simulink model "Pushbutton_to_PWMv2"  (Simulink 7.6)
settings: Solver=FixedStepDiscrete  SolverMode=SingleTasking  StartTime=0.0  StopTime=inf  FixedStep=.0001  RelTol=1e-3
undefined symbols (not defined in the file or in its folder): OC2max
libraries: simulink x16, dsPICdrivers x9, dspswit3 x1
settings Model: Creator=ij8977  LastModifiedBy=ij8977  ExtModeTrigDuration=10000
settings SolverCC: PositivePriorityOrder=on
settings OptimizationCC: OptimizeModelRefInitCode=on  LifeSpan=Inf
settings DebuggingCC: StrictBusMsg=Warning
settings RTWCC: SystemTargetFile=pic32.tlc  MakeCommand=make_CreateMPLAB  TemplateMakefile=pic32_gcc.tmf  PostCodeGenCommand=dsPIC_Compile()  Description=Embedded Target for Microchip dsPIC (real-time)  ProcessScript=pic32_make_rtw_hook
settings CodeAppCC: IgnoreCustomStorageClasses=off
settings STFCustomTargetCC: IncludeMdlTerminateFcn=off  CombineOutputUpdateFcns=on  SuppressErrorStatus=on  ERTCustomFileBanners=on  SupportContinuousTime=off  SupportNonInlinedSFcns=off  SystemTargetFile=pic32.tlc
settings ERTTargetCC: MultiwordLength=2048  ParMdlRefBuildCompliant=off  CompOptLevelCompliant=off  IncludeMdlTerminateFcn=off  SuppressErrorStatus=on  ERTFirstTimeCompliant=off  ModelStepFunctionPrototypeControlCompliant=off  CPPClassGenCompliant=off  InlinedParameterPlacement=NonHierarchical  ERTSrcFileBannerTemplate=dsPIC_code_template.cgt  ERTHdrFileBannerTemplate=dsPIC_code_template.cgt  ERTDataSrcFileTemplate=dsPIC_code_template.cgt  ERTDataHdrFileTemplate=dsPIC_code_template.cgt  ERTCustomFileTemplate=dsPIC_main.tlc  ConvertIfToSwitch=off
settings CustomProperty: DataType=string  Value=C:\PROGRA~1\MATLAB\R2010b\bin\win32\gmake

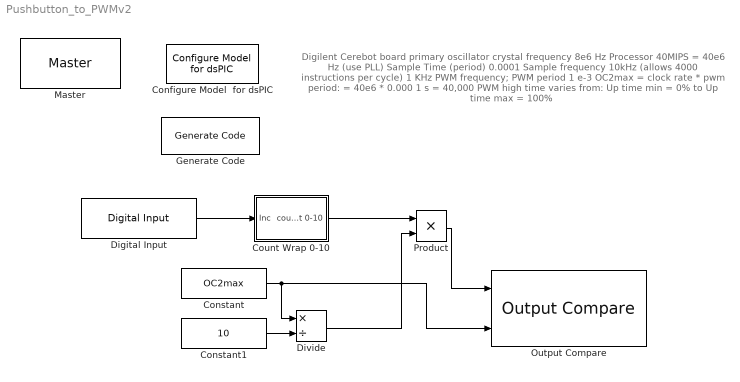
== system Pushbutton_to_PWMv2 ==
  note: Digilent Cerebot board primary oscillator crystal frequency 8e6 Hz
      | Processor 40MIPS = 40e6 Hz (use PLL)
      | Sample Time (period) 0.0001   Sample frequency 10kHz (allows 4000 instructions per cycle)
      | 1 KHz PWM frequency; PWM period 1 e-3
      | OC2max = clock rate * pwm period: = 40e6 * 0.000 1 s = 40,000
      | PWM high time varies from:
      | Up time min = 0%
      | to
      | Up time max = 100%
  Configure Model  for dsPIC : dsPICdrivers/Simulink Configuration/Configure Model  for dsPIC
  Constant : Constant  Value=OC2max  OutDataTypeStr=uint16
  Constant1 : Constant  Value=10  OutDataTypeStr=uint16
  Count Wrap 0-10 : Subsystem
  Digital Input : dsPICdrivers/Digital I//O/Digital Input  Tag=dsPIC_Digital_Input  PORT=A  Pin=[6]  SampleTime=.0001  OrderingInOutPopup=None
  Divide : Product  Inputs=*/
  Generate Code : dsPICdrivers/Simulink Configuration/Generate Code
  Master : dsPICdrivers/Master  Tag=dsPIC_MASTER  Priority=1  TimeStepType=Timer1  picType=32MX460F512L  fcy=40000000  Quartz_33f=8e6  PLLActive_33f=on  fcyDesired_33f=40e6  tmr1="[1  3999  0]"  tmr1Info="Time Step : 0.0001  ;   Error : 0%  PR1=3999"  tmr2345="[1  0  0  0]"  tmr2345cfg=[-1 -1 -1 -1]  IOautoConf=on  typePort="[ 0   0   0   0   0   0   9   0   0   0   0   0   0   0   0   0   0   0   0   0   0   0   0   0   0   0  10  10  10  10   0   0   0   0   0   0   0   0   0   0   0   0   0   0   0   0   0   0   0   7   0   0   0   0   0   0   0   0   0   0   0   0   0   0   0   0   0   0   0   0   0   0   0   0   0   0   0   0   0   0   0   0   0   0   0   0   0   0   0   0   0   0   0   0   0   0   0   0   0   0   0   0   0   0   0   0   0   0   0   0   0   0 ]"  TRIS="[ 65535  50175  65535  65533  65535  65535  65535 ]"  ADPCFG=15360  MasterBusyPort=None  MasterOverloadPort=None  FOSC=Quartz (XT - HS)  ClockSwitchMonitor=Both disabled  TempProtection_33f=TEMP_ON  FPBOR=<empty>  PWRT=disable  MCLR=<empty>  ICD=ICS_PGD1  JTAGEN=JTAGEN_OFF  PowerSave=off  OverrideFcy=off  NewFcy=1e6  PR2345="[65535  65535  65535  65535]"
  Output Compare : dsPICdrivers/Peripheral I//O/Output Compare  Tag=dsPIC_PWM_out  Priority=5  IntPriority=3  CHANNEL=[2]  Channel_UP_Down_Periode=[5]  MaxChannel=[0.001]  MaxName=' OC2max '  Precision=[15.2876]  Timer=[2]  Status=OK  SafeMarge=[0]  PortLetter=[68]  PortNumber=[1]  MaxValues=[39999]
  Product : Product  OutDataTypeStr=uint16  RndMeth=Zero
  wires:
  Digital Input/1 -> Count Wrap 0-10/1(Inc)
  Count Wrap 0-10/1(count 0-10) -> Product/1
  Constant1/1 -> Divide/2
  Constant/1 -> Divide/1, Output Compare/2
  Product/1 -> Output Compare/1
  Divide/1 -> Product/2

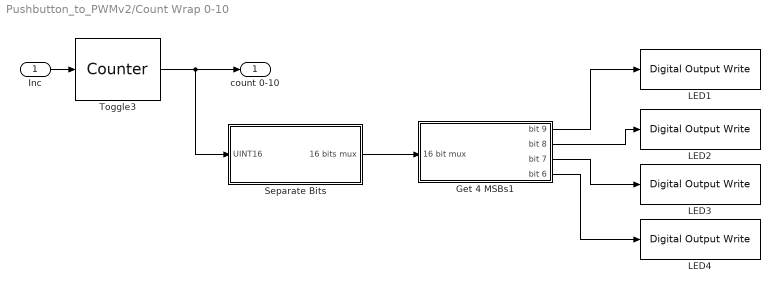
== system Pushbutton_to_PWMv2/Count Wrap 0-10 ==
  Inc : Inport
  Get 4 MSBs1 : Subsystem
  LED1 : dsPICdrivers/Digital I//O/Digital Output Write  Tag=dsPIC_Digital_Output  Priority=5  PORT=B  Pin=[10]  Simultaneous=off  OrderingInOutPopup=None
  LED2 : dsPICdrivers/Digital I//O/Digital Output Write  Tag=dsPIC_Digital_Output  Priority=5  PORT=B  Pin=[11]  Simultaneous=off  OrderingInOutPopup=None
  LED3 : dsPICdrivers/Digital I//O/Digital Output Write  Tag=dsPIC_Digital_Output  Priority=5  PORT=B  Pin=[12]  Simultaneous=off  OrderingInOutPopup=None
  LED4 : dsPICdrivers/Digital I//O/Digital Output Write  Tag=dsPIC_Digital_Output  Priority=5  PORT=B  Pin=[13]  Simultaneous=off  OrderingInOutPopup=None
  Separate Bits : Subsystem
  Toggle3 : dspswit3/Counter  Direction=Up  CountEvent=Rising edge  CounterSize=User defined  MaxCount=10  InitialCount=0  Output=Count  HitValue=10  ResetInput=off  SamplesPerFrame=1  Ts=1  CntDtype=uint16  HitDtype=Logical
  count 0-10 : Outport
  wires:
  Inc/1 -> Toggle3/1
  Get 4 MSBs1/1(bit 9) -> LED1/1
  Get 4 MSBs1/2(bit 8) -> LED2/1
  Get 4 MSBs1/3(bit 7) -> LED3/1
  Get 4 MSBs1/4(bit 6) -> LED4/1
  Separate Bits/1(16 bits mux) -> Get 4 MSBs1/1(16 bit mux)
  Toggle3/1 -> count 0-10/1, Separate Bits/1(UINT16)

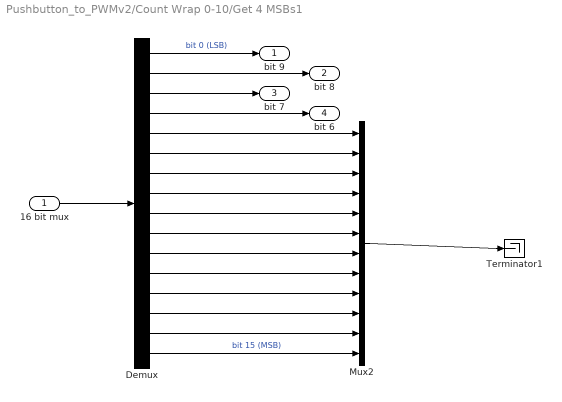
== system Pushbutton_to_PWMv2/Count Wrap 0-10/Get 4 MSBs1 ==
  16 bit mux : Inport  OutDataTypeStr=boolean
  Demux : Demux  Outputs=16
  Mux2 : Mux  Inputs=12
  Terminator1 : Terminator
  bit 9 : Outport
  bit 8 : Outport  Port=2
  bit 7 : Outport  Port=3
  bit 6 : Outport  Port=4
  wires:
  16 bit mux/1 -> Demux/1
  Mux2/1 -> Terminator1/1
  Demux/4 -> bit 6/1
  Demux/3 -> bit 7/1
  Demux/2 -> bit 8/1
  Demux/1 -> bit 9/1  "bit 0 (LSB)"
  Demux/5 -> Mux2/1
  Demux/6 -> Mux2/2
  Demux/7 -> Mux2/3
  Demux/8 -> Mux2/4
  Demux/9 -> Mux2/5
  Demux/10 -> Mux2/6
  Demux/11 -> Mux2/7
  Demux/12 -> Mux2/8
  Demux/13 -> Mux2/9
  Demux/14 -> Mux2/10
  Demux/15 -> Mux2/11
  Demux/16 -> Mux2/12  "bit 15 (MSB)"

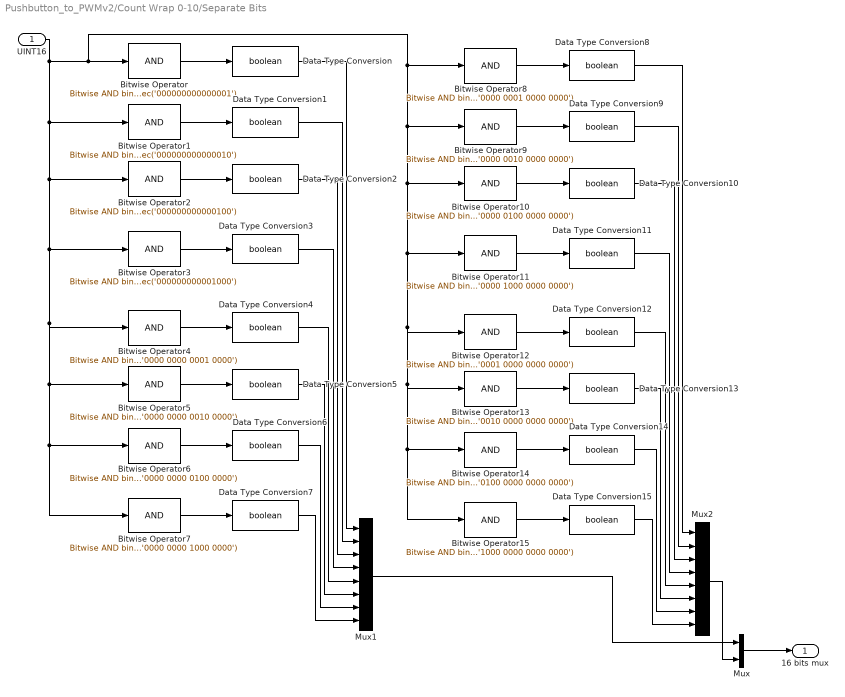
== system Pushbutton_to_PWMv2/Count Wrap 0-10/Separate Bits ==
  UINT16 : Inport
  Bitwise Operator : simulink/Logic and Bit Operations/Bitwise Operator  logicop=AND  UseBitMask=on  BitMask=bin2dec('000000000000001')  BitMaskRealWorld=Stored Integer
  Bitwise Operator1 : simulink/Logic and Bit Operations/Bitwise Operator  logicop=AND  UseBitMask=on  BitMask=bin2dec('000000000000010')  BitMaskRealWorld=Stored Integer
  Bitwise Operator10 : simulink/Logic and Bit Operations/Bitwise Operator  logicop=AND  UseBitMask=on  BitMask=bin2dec('0000 0100 0000 0000')  BitMaskRealWorld=Stored Integer
  Bitwise Operator11 : simulink/Logic and Bit Operations/Bitwise Operator  logicop=AND  UseBitMask=on  BitMask=bin2dec('0000 1000 0000 0000')  BitMaskRealWorld=Stored Integer
  Bitwise Operator12 : simulink/Logic and Bit Operations/Bitwise Operator  logicop=AND  UseBitMask=on  BitMask=bin2dec('0001 0000 0000 0000')  BitMaskRealWorld=Stored Integer
  Bitwise Operator13 : simulink/Logic and Bit Operations/Bitwise Operator  logicop=AND  UseBitMask=on  BitMask=bin2dec('0010 0000 0000 0000')  BitMaskRealWorld=Stored Integer
  Bitwise Operator14 : simulink/Logic and Bit Operations/Bitwise Operator  logicop=AND  UseBitMask=on  BitMask=bin2dec('0100 0000 0000 0000')  BitMaskRealWorld=Stored Integer
  Bitwise Operator15 : simulink/Logic and Bit Operations/Bitwise Operator  logicop=AND  UseBitMask=on  BitMask=bin2dec('1000 0000 0000 0000')  BitMaskRealWorld=Stored Integer
  Bitwise Operator2 : simulink/Logic and Bit Operations/Bitwise Operator  logicop=AND  UseBitMask=on  BitMask=bin2dec('000000000000100')  BitMaskRealWorld=Stored Integer
  Bitwise Operator3 : simulink/Logic and Bit Operations/Bitwise Operator  logicop=AND  UseBitMask=on  BitMask=bin2dec('000000000001000')  BitMaskRealWorld=Stored Integer
  Bitwise Operator4 : simulink/Logic and Bit Operations/Bitwise Operator  logicop=AND  UseBitMask=on  BitMask=bin2dec('0000 0000 0001 0000')  BitMaskRealWorld=Stored Integer
  Bitwise Operator5 : simulink/Logic and Bit Operations/Bitwise Operator  logicop=AND  UseBitMask=on  BitMask=bin2dec('0000 0000 0010 0000')  BitMaskRealWorld=Stored Integer
  Bitwise Operator6 : simulink/Logic and Bit Operations/Bitwise Operator  logicop=AND  UseBitMask=on  BitMask=bin2dec('0000 0000 0100 0000')  BitMaskRealWorld=Stored Integer
  Bitwise Operator7 : simulink/Logic and Bit Operations/Bitwise Operator  logicop=AND  UseBitMask=on  BitMask=bin2dec('0000 0000 1000 0000')  BitMaskRealWorld=Stored Integer
  Bitwise Operator8 : simulink/Logic and Bit Operations/Bitwise Operator  logicop=AND  UseBitMask=on  BitMask=bin2dec('0000 0001 0000 0000')  BitMaskRealWorld=Stored Integer
  Bitwise Operator9 : simulink/Logic and Bit Operations/Bitwise Operator  logicop=AND  UseBitMask=on  BitMask=bin2dec('0000 0010 0000 0000')  BitMaskRealWorld=Stored Integer
  Data Type Conversion{,1..15} (16 alike) : DataTypeConversion  OutDataTypeStr=boolean
  Mux : Mux  Inputs=2
  Mux1 : Mux  Inputs=8
  Mux2 : Mux  Inputs=8
  16 bits mux : Outport
  wires:
  Mux2/1 -> Mux/2
  Bitwise Operator15/1 -> Data Type Conversion15/1
  Bitwise Operator14/1 -> Data Type Conversion14/1
  Bitwise Operator13/1 -> Data Type Conversion13/1
  Bitwise Operator12/1 -> Data Type Conversion12/1
  Bitwise Operator11/1 -> Data Type Conversion11/1
  Bitwise Operator10/1 -> Data Type Conversion10/1
  Bitwise Operator9/1 -> Data Type Conversion9/1
  Data Type Conversion15/1 -> Mux2/8
  Data Type Conversion14/1 -> Mux2/7
  Data Type Conversion13/1 -> Mux2/6
  Data Type Conversion12/1 -> Mux2/5
  Data Type Conversion11/1 -> Mux2/4
  Data Type Conversion10/1 -> Mux2/3
  Data Type Conversion9/1 -> Mux2/2
  Data Type Conversion8/1 -> Mux2/1
  Bitwise Operator8/1 -> Data Type Conversion8/1
  Bitwise Operator7/1 -> Data Type Conversion7/1
  Bitwise Operator6/1 -> Data Type Conversion6/1
  Bitwise Operator5/1 -> Data Type Conversion5/1
  Bitwise Operator4/1 -> Data Type Conversion4/1
  Bitwise Operator3/1 -> Data Type Conversion3/1
  Bitwise Operator2/1 -> Data Type Conversion2/1
  Bitwise Operator1/1 -> Data Type Conversion1/1
  Mux/1 -> 16 bits mux/1
  Mux1/1 -> Mux/1
  Data Type Conversion7/1 -> Mux1/8
  Data Type Conversion6/1 -> Mux1/7
  Data Type Conversion5/1 -> Mux1/6
  Data Type Conversion4/1 -> Mux1/5
  Data Type Conversion3/1 -> Mux1/4
  Data Type Conversion2/1 -> Mux1/3
  Data Type Conversion1/1 -> Mux1/2
  Data Type Conversion/1 -> Mux1/1
  Bitwise Operator/1 -> Data Type Conversion/1
  UINT16/1 -> Bitwise Operator8/1, Bitwise Operator9/1, Bitwise Operator10/1, Bitwise Operator11/1, Bitwise Operator12/1, Bitwise Operator13/1, Bitwise Operator14/1, Bitwise Operator15/1, Bitwise Operator/1, Bitwise Operator2/1, Bitwise Operator3/1, Bitwise Operator4/1, Bitwise Operator5/1, Bitwise Operator6/1, Bitwise Operator7/1, Bitwise Operator1/1
